simulink model "s_b4a4x1kf"  (R2018a)
settings: Solver=VariableStepDiscrete  StartTime=0.0  StopTime=1  RelTol=1e-3
undefined symbols (not defined in the file): fft_stages, n_bits_ants, n_bits_xengs
libraries: xbsIndex_r4 x22055, xbsReplacements_r4 x30, casper_library_misc x29, casper_library_scopes x15, xps_library x4
(part 89 of 227)

== system s_b4a4x1kf/sys3/vacc/vacc_time ==
  note: If we're going to relock,
      | lock two accs ahead.
      | (give VACCs chance to reset)
  note: If we were armed and somehow missed the
      | trigger, then re-arm.
      |
      | If we're waiting for a timestamp more than 2 accs ahead
      | (rew) of incoming timestamps, also re-arm.
      |
      | If an error occurs inside the VACC, also re-arm.
  note: If we detected an error,
      | wait 'till we've caught up to the incoming timestamp,
      | then rearm.
  note: fast-forward if we're
      | behind the incoming
      | timestamp.
  note: Rewind our record if we're more than
      | 2 accumulations ahead of incoming
      | timestampls.
  timestamp_in : Inport
  acc_len : Inport  Port=2
  valid_in : Inport  Port=3
  rb_done : Inport  Port=4
  arm : Inport  Port=5
  load_time : Inport  Port=6
  immediate : Inport  Port=7
  ext_err : Inport  Port=8
  AddSub : xbsIndex_r4/AddSub  mode=Subtraction  use_carryin=off  use_carryout=off  en=off  latency=1  precision=User Defined  arith_type=Unsigned  n_bits=timestamp_bits  bin_pt=0  quantization=Truncate  overflow=Wrap  use_behavioral_HDL=off  hw_selection=Fabric  pipelined=off  dbl_ovrd=off  block_type=addsub
  AddSub1 : xbsIndex_r4/AddSub  mode=Addition or Subtraction  use_carryin=off  use_carryout=off  en=on  latency=1  precision=User Defined  arith_type=Unsigned  n_bits=timestamp_bits  bin_pt=0  quantization=Truncate  overflow=Wrap  use_behavioral_HDL=on  hw_selection=Fabric  pipelined=off  dbl_ovrd=off  block_type=addsub
  AddSub2 : xbsIndex_r4/AddSub  mode=Addition  use_carryin=off  use_carryout=off  en=off  latency=1  precision=User Defined  arith_type=Unsigned  n_bits=timestamp_bits  bin_pt=0  quantization=Truncate  overflow=Wrap  use_behavioral_HDL=off  hw_selection=Fabric  pipelined=off  dbl_ovrd=off  block_type=addsub
  AddSub4 : xbsIndex_r4/AddSub  mode=Addition  use_carryin=off  use_carryout=off  en=off  latency=1  precision=User Defined  arith_type=Unsigned  n_bits=timestamp_bits  bin_pt=0  quantization=Truncate  overflow=Wrap  use_behavioral_HDL=off  hw_selection=Fabric  pipelined=off  dbl_ovrd=off  block_type=addsub
  Constant1 : xbsIndex_r4/Constant  const=0  gui_display_data_type=Fixed-point  arith_type=Unsigned  n_bits=1  bin_pt=0  preci_type=Single  exp_width=8  frac_width=24  explicit_period=on  period=1  equ=P=C  opselect=C  inp2=PCIN>>17  opr=+  inp1=P  carry=CIN  dbl_ovrd=off  block_type=constant
  Delay{7..10,13..14,23,26..29,32} (12 alike) : xbsIndex_r4/Delay  rst=off  infoeditControl=Selection of Reset will increase slice count due to use of real FFs and instead of SRLs  en=off  latency=1  reg_retiming=on  dbl_ovrd=off  block_type=delay
      Delay10 settings: infoedit=Hardware notes: A delay line is a chain, each link of which is an SRL16 or SRL32 followed by a flip-flop.
      Delay13 settings: infoedit=Hardware notes: A delay line is a chain, each link of which is an SRL16 or SRL32 followed by a flip-flop.
      Delay14 settings: infoedit=Hardware notes: A delay line is a chain, each link of which is an SRL16 or SRL32 followed by a flip-flop.
      Delay23 settings: infoedit=Hardware notes: A delay line is a chain, each link of which is an SRL16 or SRL32 followed by a flip-flop.
      Delay26 settings: infoedit=Hardware notes: A delay line is a chain, each link of which is an SRL16 or SRL32 followed by a flip-flop.
      Delay27 settings: infoedit=Hardware notes: A delay line is a chain, each link of which is an SRL16 or SRL32 followed by a flip-flop.
      Delay28 settings: infoedit=Hardware notes: A delay line is a chain, each link of which is an SRL16 or SRL32 followed by a flip-flop.
      Delay32 settings: infoedit=Hardware notes: A delay line is a chain, each link of which is an SRL16 or SRL32 followed by a flip-flop.
      Delay7 settings: infoedit=Hardware notes: A delay line is a chain, each link of which is an SRL16 or SRL32 followed by a flip-flop.
      Delay9 settings: infoedit=Hardware notes: A delay line is a chain, each link of which is an SRL16 or SRL32 followed by a flip-flop.
  Delay{15..16,19..22,30} (7 alike) : xbsIndex_r4/Delay  rst=off  infoeditControl=Selection of Reset will increase slice count due to use of real FFs and instead of SRLs  en=off  latency=2  reg_retiming=on  dbl_ovrd=off  block_type=delay
      settings: infoedit=Hardware notes: A delay line is a chain, each link of which is an SRL16 or SRL32 followed by a flip-flop.
  FIFO : xbsIndex_r4/FIFO  mem_type=Distributed RAM  performance_options=First_Word_Fall_Through  embedded_registers=off  depth=16  percent_nbits=1  rst=on  rst_latency=1  en=off  use_dcount=off  use_percent_full_port=off  use_almost_empty=off  almost_empty_thresh=2  use_almost_full=off  use_rd_rst_busy=off  use_wr_rst_busy=off  almost_full_thresh=14  explicit_period=off  dbl_ovrd=off  block_type=fifo
  Inverter{,1..3} (4 alike) : xbsIndex_r4/Inverter  en=off  latency=0  dbl_ovrd=off  block_type=inv
  Logical : xbsIndex_r4/Logical  logical_function=OR  inputs=3  en=off  latency=0  precision=Full  arith_type=Unsigned  n_bits=16  bin_pt=0  align_bp=on  dbl_ovrd=off  block_type=logical
  Logical{1,7,12..13} (4 alike) : xbsIndex_r4/Logical  logical_function=AND  inputs=2  en=off  latency=0  precision=Full  arith_type=Unsigned  n_bits=16  bin_pt=0  align_bp=on  dbl_ovrd=off  block_type=logical
  Logical10 : xbsIndex_r4/Logical  logical_function=OR  inputs=3  en=off  latency=0  precision=Full  arith_type=Unsigned  n_bits=16  bin_pt=0  align_bp=on  dbl_ovrd=off  block_type=logical
  Logical{4..5,9,11} (4 alike) : xbsIndex_r4/Logical  logical_function=OR  inputs=2  en=off  latency=0  precision=Full  arith_type=Unsigned  n_bits=16  bin_pt=0  align_bp=on  dbl_ovrd=off  block_type=logical
  Logical2 : xbsIndex_r4/Logical  logical_function=OR  inputs=4  en=off  latency=0  precision=Full  arith_type=Unsigned  n_bits=16  bin_pt=0  align_bp=on  dbl_ovrd=off  block_type=logical
  Logical3 : xbsIndex_r4/Logical  logical_function=AND  inputs=3  en=off  latency=0  precision=Full  arith_type=Unsigned  n_bits=16  bin_pt=0  align_bp=on  dbl_ovrd=off  block_type=logical
  Mux : xbsIndex_r4/Mux  inputs=2  en=off  latency=1  precision=Full  arith_type=Unsigned  n_bits=16  bin_pt=14  quantization=Truncate  overflow=Wrap  dbl_ovrd=off  block_type=mux
  Register{1..3,5} (4 alike) : xbsIndex_r4/Register  init=0  rst=off  en=on  dbl_ovrd=off  block_type=register
  Register4 : xbsIndex_r4/Register  init=0  rst=on  en=on  dbl_ovrd=off  block_type=register
  Relational : xbsIndex_r4/Relational  mode=a!=b  op_type=Bool  en=off  latency=1  dbl_ovrd=off  block_type=relational
  Relational1 : xbsIndex_r4/Relational  mode=a>b  op_type=Bool  en=off  latency=1  dbl_ovrd=off  block_type=relational
  Relational2 : xbsIndex_r4/Relational  mode=a=b  op_type=Bool  en=off  latency=1  dbl_ovrd=off  block_type=relational
      settings: block_version=10.1.3
  Relational3 : xbsIndex_r4/Relational  mode=a=b  op_type=Bool  en=off  latency=1  dbl_ovrd=off  block_type=relational
      settings: block_version=10.1.3
  Relational4 : xbsIndex_r4/Relational  mode=a!=b  op_type=Bool  en=off  latency=1  dbl_ovrd=off  block_type=relational
  Relational5 : xbsIndex_r4/Relational  mode=a<b  op_type=Bool  en=off  latency=1  dbl_ovrd=off  block_type=relational
  Relational6 : xbsIndex_r4/Relational  mode=a>b  op_type=Bool  en=off  latency=1  dbl_ovrd=off  block_type=relational
  Shift : xbsIndex_r4/Shift  shift_dir=Left  shift_bits=1  en=off  latency=0  precision=Full  arith_type="Signed  (2's comp)"  n_bits=16  bin_pt=14  quantization=Truncate  overflow=Wrap  dbl_ovrd=off  block_type=shift
  Shift2 : xbsIndex_r4/Shift  shift_dir=Left  shift_bits=1  en=off  latency=0  precision=Full  arith_type="Signed  (2's comp)"  n_bits=16  bin_pt=14  quantization=Truncate  overflow=Wrap  dbl_ovrd=off  block_type=shift
  armed_reg : xbsIndex_r4/Register  init=0  rst=on  en=on  dbl_ovrd=off  block_type=register
  edge_detect1 : Subsystem  mask(edge_detect){edge=Rising, polarity=Active High, x_in=[0 0.08 0.08 0.16 0.16 0.24 0.24 0.32 0.32 0.4], y_in=[-1 -1  1  1  1  1  1  1  1  1], x_out=[0.6 0.68 0.68 0.76 0.76 0.84 0.84 0.92 0.92 1], y_out=[-1 -1  1  1 -1 -1 -1 -1 -1 -1]}
      mask prompts: edge "Edge Type"; polarity "Output Polarity"; x_in "Input X Positions"; y_in "Input Y Positions"; x_out "Output X Positions"; y_out "Output Y Positions"
      mask help: Output is active for one-cycle after each edge of the specified type (i.e. rising, falling or both).
      mask init: same as s_b4a4x1kf/edge_detect
      settings: AttributesFormatString=|
      | rising edges
      | active high
      mask Help: Output is active for one-cycle after each edge of the specified type (i.e. rising, falling, or both).  Latency is zero.
      mask TypeOptions edge: Rising | Falling | Both
      mask TypeOptions polarity: Active High | Active Low
      mask Display:
      | plot(x_in_num,0.5+y_in_num*0.2);
      | plot(x_out_num,0.5+y_out_num*0.2);
  edge_detect2 : Subsystem  mask(edge_detect){edge=Rising, polarity=Active High, x_in=[0 0.08 0.08 0.16 0.16 0.24 0.24 0.32 0.32 0.4], y_in=[-1 -1  1  1  1  1  1  1  1  1], x_out=[0.6 0.68 0.68 0.76 0.76 0.84 0.84 0.92 0.92 1], y_out=[-1 -1  1  1 -1 -1 -1 -1 -1 -1]}
      mask prompts: edge "Edge Type"; polarity "Output Polarity"; x_in "Input X Positions"; y_in "Input Y Positions"; x_out "Output X Positions"; y_out "Output Y Positions"
      mask help: Output is active for one-cycle after each edge of the specified type (i.e. rising, falling or both).
      mask init: same as s_b4a4x1kf/edge_detect
      settings: AttributesFormatString=|
      | rising edges
      | active high
      mask Help: Output is active for one-cycle after each edge of the specified type (i.e. rising, falling, or both).  Latency is zero.
      mask TypeOptions edge: Rising | Falling | Both
      mask TypeOptions polarity: Active High | Active Low
      mask Display:
      | plot(x_in_num,0.5+y_in_num*0.2);
      | plot(x_out_num,0.5+y_out_num*0.2);
  edge_detect3 : Subsystem  mask(edge_detect){edge=Rising, polarity=Active High, x_in=[0 0.08 0.08 0.16 0.16 0.24 0.24 0.32 0.32 0.4], y_in=[-1 -1  1  1  1  1  1  1  1  1], x_out=[0.6 0.68 0.68 0.76 0.76 0.84 0.84 0.92 0.92 1], y_out=[-1 -1  1  1 -1 -1 -1 -1 -1 -1]}
      mask prompts: edge "Edge Type"; polarity "Output Polarity"; x_in "Input X Positions"; y_in "Input Y Positions"; x_out "Output X Positions"; y_out "Output Y Positions"
      mask help: Output is active for one-cycle after each edge of the specified type (i.e. rising, falling or both).
      mask init: same as s_b4a4x1kf/edge_detect
      settings: AttributesFormatString=|
      | rising edges
      | active high
      mask Help: Output is active for one-cycle after each edge of the specified type (i.e. rising, falling, or both).  Latency is zero.
      mask TypeOptions edge: Rising | Falling | Both
      mask TypeOptions polarity: Active High | Active Low
      mask Display:
      | plot(x_in_num,0.5+y_in_num*0.2);
      | plot(x_out_num,0.5+y_out_num*0.2);
  edge_detect4 : Subsystem  mask(edge_detect){edge=Rising, polarity=Active High, x_in=[0 0.08 0.08 0.16 0.16 0.24 0.24 0.32 0.32 0.4], y_in=[-1 -1  1  1  1  1  1  1  1  1], x_out=[0.6 0.68 0.68 0.76 0.76 0.84 0.84 0.92 0.92 1], y_out=[-1 -1  1  1 -1 -1 -1 -1 -1 -1]}
      mask prompts: edge "Edge Type"; polarity "Output Polarity"; x_in "Input X Positions"; y_in "Input Y Positions"; x_out "Output X Positions"; y_out "Output Y Positions"
      mask help: Output is active for one-cycle after each edge of the specified type (i.e. rising, falling or both).
      mask init: same as s_b4a4x1kf/edge_detect
      settings: AttributesFormatString=|
      | rising edges
      | active high
      mask Help: Output is active for one-cycle after each edge of the specified type (i.e. rising, falling, or both).  Latency is zero.
      mask TypeOptions edge: Rising | Falling | Both
      mask TypeOptions polarity: Active High | Active Low
      mask Display:
      | plot(x_in_num,0.5+y_in_num*0.2);
      | plot(x_out_num,0.5+y_out_num*0.2);
  edge_detect5 : Subsystem  mask(edge_detect){edge=Rising, polarity=Active High, x_in=[0 0.08 0.08 0.16 0.16 0.24 0.24 0.32 0.32 0.4], y_in=[-1 -1  1  1  1  1  1  1  1  1], x_out=[0.6 0.68 0.68 0.76 0.76 0.84 0.84 0.92 0.92 1], y_out=[-1 -1  1  1 -1 -1 -1 -1 -1 -1]}
      mask prompts: edge "Edge Type"; polarity "Output Polarity"; x_in "Input X Positions"; y_in "Input Y Positions"; x_out "Output X Positions"; y_out "Output Y Positions"
      mask help: Output is active for one-cycle after each edge of the specified type (i.e. rising, falling or both).
      mask init: same as s_b4a4x1kf/edge_detect
      settings: AttributesFormatString=|
      | rising edges
      | active high
      mask Help: Output is active for one-cycle after each edge of the specified type (i.e. rising, falling, or both).  Latency is zero.
      mask TypeOptions edge: Rising | Falling | Both
      mask TypeOptions polarity: Active High | Active Low
      mask Display:
      | plot(x_in_num,0.5+y_in_num*0.2);
      | plot(x_out_num,0.5+y_out_num*0.2);
  edge_detect6 : Subsystem  mask(edge_detect){edge=Rising, polarity=Active High, x_in=[0 0.08 0.08 0.16 0.16 0.24 0.24 0.32 0.32 0.4], y_in=[-1 -1  1  1  1  1  1  1  1  1], x_out=[0.6 0.68 0.68 0.76 0.76 0.84 0.84 0.92 0.92 1], y_out=[-1 -1  1  1 -1 -1 -1 -1 -1 -1]}
      mask prompts: edge "Edge Type"; polarity "Output Polarity"; x_in "Input X Positions"; y_in "Input Y Positions"; x_out "Output X Positions"; y_out "Output Y Positions"
      mask help: Output is active for one-cycle after each edge of the specified type (i.e. rising, falling or both).
      mask init: same as s_b4a4x1kf/edge_detect
      settings: AttributesFormatString=|
      | rising edges
      | active high
      mask Help: Output is active for one-cycle after each edge of the specified type (i.e. rising, falling, or both).  Latency is zero.
      mask TypeOptions edge: Rising | Falling | Both
      mask TypeOptions polarity: Active High | Active Low
      mask Display:
      | plot(x_in_num,0.5+y_in_num*0.2);
      | plot(x_out_num,0.5+y_out_num*0.2);
  edge_detect7 : Subsystem  mask(edge_detect){edge=Both, polarity=Active High, x_in=[0 0.08 0.08 0.16 0.16 0.24 0.24 0.32 0.32 0.4], y_in=[-1 -1  1  1  1  1  1  1  1  1], x_out=[0.6 0.68 0.68 0.76 0.76 0.84 0.84 0.92 0.92 1], y_out=[-1 -1  1  1 -1 -1 -1 -1 -1 -1]}
      mask prompts: edge "Edge Type"; polarity "Output Polarity"; x_in "Input X Positions"; y_in "Input Y Positions"; x_out "Output X Positions"; y_out "Output Y Positions"
      mask help: Output is active for one-cycle after each edge of the specified type (i.e. rising, falling or both).
      mask init: same as s_b4a4x1kf/edge_detect
      settings: AttributesFormatString=|
      | both edges
      | active high
      mask Help: Output is active for one-cycle after each edge of the specified type (i.e. rising, falling, or both).  Latency is zero.
      mask TypeOptions edge: Rising | Falling | Both
      mask TypeOptions polarity: Active High | Active Low
      mask Display:
      | plot(x_in_num,0.5+y_in_num*0.2);
      | plot(x_out_num,0.5+y_out_num*0.2);
  segment : Subsystem
  timestamp_out : Outport
  armed : Outport  Port=2
  acc_start : Outport  Port=3
  ts_err : Outport  Port=4
  wires:
  armed_reg/1 -> [armed]
  rb_done/1 -> edge_detect1/1(in)
  Register2/1 -> AddSub/2
  AddSub/1 -> Relational/1, Relational4/1
  [acc_len] -> Relational/2
  Delay7/1 -> AddSub1/2
  [armed] -> Delay20/1
  acc_len/1 -> [acc_len]
  [acc_len] -> segment/3(acc_len)
  [acc_len] -> Delay7/1
  Logical/1 -> armed_reg/2
  arm/1 -> edge_detect3/1(in)
  load_time/1 -> Register3/1
  Register3/1 -> [ext_load_time_latched], Relational2/2
  immediate/1 -> Delay32/1
  Relational2/1 -> edge_detect4/1(in)
  Delay8/1 -> edge_detect5/1(in)
  edge_detect4/1(out) -> Logical/1
  timestamp_in/1 -> Delay10/1, Relational3/1, Relational2/1
  [armed] -> segment/1(arm)
  [armed] -> armed/1
  [acc_start] -> Logical2/1
  Relational1/1 -> [ffwd]
  [ffwd] -> Logical2/2
  valid_in/1 -> Delay9/1
  [valid_in] -> segment/2(valid)
  Register4/1 -> [latched_err]
  [ffwd] -> Inverter/1
  [latched_err] -> Logical3/1
  Inverter/1 -> Logical3/2
  Relational3/1 -> edge_detect2/1(in)
  edge_detect2/1(out) -> Logical/2
  edge_detect5/1(out) -> Logical/3
  Logical4/1 -> [rearm], armed_reg/3, armed_reg/1
  [ext_arm] -> Logical4/2
  [relock_arm] -> edge_detect6/1(in)
  edge_detect6/1(out) -> Logical4/1
  [relock_ts] -> Mux/2
  Mux/1 -> AddSub1/1
  [ext_load_time_latched] -> Mux/3
  Inverter1/1 -> Logical3/3
  Logical11/1 -> Register1/2
  Delay9/1 -> Delay13/1
  Delay10/1 -> Delay14/1
  Delay13/1 -> [valid_in]
  Delay14/1 -> [ts_in]
  [ts_in] -> Delay15/1
  [valid_in] -> Delay16/1
  [armed] -> Delay22/1
  Delay19/1 -> Register1/1
  segment/1(acc_start) -> [acc_start]
  [ext_arm] -> Delay26/1
  [ext_arm] -> Mux/1
  Delay20/1 -> Logical11/2, Delay21/1
  Delay21/1 -> Logical5/2
  Logical5/1 -> Register2/2
  [acc_start] -> Logical5/1
  [acc_start] -> Logical11/1
  FIFO/1 -> [ts_out], timestamp_out/1
  edge_detect1/1(out) -> [rb_done]
  [ts_in] -> Delay19/1
  edge_detect3/1(out) -> Register3/2, Delay27/1
  [acc_start] -> acc_start/1
  [rb_done] -> FIFO/3
  [acc_start] -> Delay28/1
  [ts_in] -> Delay23/1
  [armed] -> FIFO/4
  Delay23/1 -> FIFO/1
  Delay28/1 -> FIFO/2
  Constant1/1 -> Relational4/2
  Relational/1 -> Logical1/1
  Relational4/1 -> Logical1/2
  Logical1/1 -> [ts_err]
  Register1/1 -> Register2/1, Delay29/1
  Delay29/1 -> AddSub/1
  Logical2/1 -> AddSub1/4
  Relational5/1 -> [rew]
  [rew] -> Logical2/4
  [rew] -> AddSub1/3
  [relock_ts] -> Relational5/2
  [ts_in] -> AddSub2/1
  AddSub2/1 -> Relational5/1
  [acc_len] -> Shift/1
  Shift/1 -> AddSub2/2
  Delay30/1 -> ts_err/1
  [rew] -> Inverter1/1
  [latched_relock_ts] -> Relational3/2
  Logical3/1 -> [relock_arm]
  Logical10/1 -> Register4/3, Register4/1
  [ts_err] -> Logical12/1
  [armed] -> Inverter2/1
  Inverter2/1 -> Logical12/2
  Logical12/1 -> Logical10/2
  [rearm] -> Register4/2
  [relock_ts] -> Relational1/2
  [ts_in] -> Relational1/1
  [latched_relock_ts] -> Relational6/2
  [ts_in] -> Relational6/1
  AddSub1/1 -> [relock_ts]
  [relock_arm] -> Register5/2
  Register5/1 -> [latched_relock_ts]
  Shift2/1 -> AddSub4/2
  [relock_ts] -> AddSub4/1
  [acc_len] -> Shift2/1
  AddSub4/1 -> Register5/1
  Logical7/1 -> Logical10/1
  [armed] -> Logical7/2
  Relational6/1 -> Logical9/1
  Logical9/1 -> Logical7/1
  [rew] -> Logical9/2
  Delay26/1 -> Logical2/3
  Delay27/1 -> [ext_arm]
  Delay32/1 -> Delay8/1
  Inverter3/1 -> Logical13/2
  [armed] -> Inverter3/1
  [ext_err] -> Logical13/1
  Logical13/1 -> Logical10/3
  ext_err/1 -> [ext_err]
  [latched_err] -> edge_detect7/1(in)
  edge_detect7/1(out) -> Delay30/1

== system s_b4a4x1kf/sys3/vacc_tvg0/bus_replicate1 ==
  in : Inport
  bussify : Subsystem  mask(bus_create){inputNum=8}
      mask prompts: inputNum "Number of inputs:"
      mask init:
      | bus_create_init(gcb,...
      |     'inputNum', inputNum);
  out : Outport
  wires:
  in/1 -> bussify/1(in1), bussify/2(in2), bussify/3(in3), bussify/4(in4), bussify/5(in5), bussify/6(in6), bussify/7(in7), bussify/8(in8)
  bussify/1(bus_out) -> out/1

== system s_b4a4x1kf/sys3/vacc_tvg0/bus_replicate2 ==
  in : Inport
  bussify : Subsystem  mask(bus_create){inputNum=8}
      mask prompts: inputNum "Number of inputs:"
      mask init:
      | bus_create_init(gcb,...
      |     'inputNum', inputNum);
  out : Outport
  wires:
  in/1 -> bussify/1(in1), bussify/2(in2), bussify/3(in3), bussify/4(in4), bussify/5(in5), bussify/6(in6), bussify/7(in7), bussify/8(in8)
  bussify/1(bus_out) -> out/1

== system s_b4a4x1kf/sys3/vacc_tvg0/edge_detect ==
  in : Inport
  Delay : xbsIndex_r4/Delay  rst=off  infoeditControl=Selection of Reset will increase slice count due to use of real FFs and instead of SRLs  en=off  latency=1  reg_retiming=off  dbl_ovrd=off  block_type=delay
      settings: xl_area=[0, 0, 0, 0, 0, 0, 0]
  Inverter : xbsIndex_r4/Inverter  en=off  latency=0  dbl_ovrd=off  block_type=inv
      settings: xl_area=[0, 0, 0, 0, 0, 0, 0]
  edge_op : xbsIndex_r4/Logical  logical_function=NOR  inputs=2  en=off  latency=0  precision=Full  arith_type=Unsigned  n_bits=8  bin_pt=2  align_bp=on  dbl_ovrd=off  block_type=logical
      settings: xl_area=[0, 0, 0, 0, 0, 0, 0]
  out : Outport
  wires:
  Delay/1 -> edge_op/2
  in/1 -> Delay/1, Inverter/1
  edge_op/1 -> out/1
  Inverter/1 -> edge_op/1

== system s_b4a4x1kf/sys3/vacc_tvg0/edge_detect4 ==
  in : Inport
  Delay : xbsIndex_r4/Delay  rst=off  infoeditControl=Selection of Reset will increase slice count due to use of real FFs and instead of SRLs  en=off  latency=1  reg_retiming=on  dbl_ovrd=off  block_type=delay
      settings: xl_area=[0, 0, 0, 0, 0, 0, 0]
  Inverter : xbsIndex_r4/Inverter  en=off  latency=0  dbl_ovrd=off  block_type=inv
      settings: xl_area=[0, 0, 0, 0, 0, 0, 0]
  edge_op : xbsIndex_r4/Logical  logical_function=NOR  inputs=2  en=off  latency=0  precision=Full  arith_type=Unsigned  n_bits=8  bin_pt=2  align_bp=on  dbl_ovrd=off  block_type=logical
      settings: xl_area=[0, 0, 0, 0, 0, 0, 0]
  out : Outport
  wires:
  Inverter/1 -> edge_op/1
  edge_op/1 -> out/1
  in/1 -> Inverter/1, Delay/1
  Delay/1 -> edge_op/2

== system s_b4a4x1kf/sys3/vacc_tvg0/generate_pulses ==
  run : Inport
  num_pulses : Inport  Port=2
  num_per_group : Inport  Port=3
  group period : Inport  Port=4
  Constant : xbsIndex_r4/Constant  const=777777  gui_display_data_type=Fixed-point  arith_type=Unsigned  n_bits=20  bin_pt=0  preci_type=Single  exp_width=8  frac_width=24  explicit_period=on  period=1  equ=P=C  opselect=C  inp2=PCIN>>17  opr=+  inp1=P  carry=CIN  dbl_ovrd=off  block_type=constant
  Gateway Out{1..8} (8 alike) : xbsIndex_r4/Gateway Out  inherit_from_input=off  hdl_port=off  rows=1  columns=1  UseAsDAC=off  DACChannel='1'  interface=None  automatic_assignment=on  address_offset=hex2dec('00')  intf_name=''  intf_description=''  timing_constraint=None  locs_specified=off  LOCs={}  io_standard={}  block_type=gatewayout
      settings: infoedit="Gateway out block.  Converts Xilinx fixed point inputs into ouputs of type Simulink integer, double, or fixed point.<P><P>Hardware notes:  In hardware these blocks become top level output ports or are discarded, depending on how they are configured."  xl_area=[0, 0, 0, 0, 0, 0, 0]  block_version=10.1.3
  Inverter : xbsIndex_r4/Inverter  en=off  latency=0  dbl_ovrd=off  block_type=inv
  Logical1 : xbsIndex_r4/Logical  logical_function=AND  inputs=2  en=off  latency=0  precision=Full  arith_type=Unsigned  n_bits=8  bin_pt=2  align_bp=on  dbl_ovrd=off  block_type=logical
      settings: xl_area=[0, 0, 0, 0, 0, 0, 0]
  Logical2 : xbsIndex_r4/Logical  logical_function=AND  inputs=3  en=off  latency=0  precision=Full  arith_type=Unsigned  n_bits=8  bin_pt=2  align_bp=on  dbl_ovrd=off  block_type=logical
      settings: xl_area=[0, 0, 0, 0, 0, 0, 0]
  Logical3 : xbsIndex_r4/Logical  logical_function=AND  inputs=3  en=off  latency=0  precision=Full  arith_type=Unsigned  n_bits=8  bin_pt=2  align_bp=on  dbl_ovrd=off  block_type=logical
      settings: xl_area=[0, 0, 0, 0, 0, 0, 0]
  Logical4 : xbsIndex_r4/Logical  logical_function=OR  inputs=2  en=off  latency=0  precision=Full  arith_type=Unsigned  n_bits=8  bin_pt=2  align_bp=off  dbl_ovrd=off  block_type=logical
      settings: xl_area=[0, 0, 0, 0, 0, 0, 0]
  Logical5 : xbsIndex_r4/Logical  logical_function=OR  inputs=2  en=off  latency=0  precision=Full  arith_type=Unsigned  n_bits=8  bin_pt=2  align_bp=on  dbl_ovrd=off  block_type=logical
      settings: xl_area=[0, 0, 0, 0, 0, 0, 0]
  Logical6 : xbsIndex_r4/Logical  logical_function=AND  inputs=2  en=off  latency=0  precision=Full  arith_type=Unsigned  n_bits=8  bin_pt=2  align_bp=on  dbl_ovrd=off  block_type=logical
      settings: xl_area=[0, 0, 0, 0, 0, 0, 0]
  Relational : xbsIndex_r4/Relational  mode=a>=b  op_type=Bool  en=off  latency=0  dbl_ovrd=off  block_type=relational
      settings: xl_area=[0, 0, 0, 0, 0, 0, 0]  block_version=10.1.3
  Relational1 : xbsIndex_r4/Relational  mode=a=b  op_type=Bool  en=off  latency=0  dbl_ovrd=off  block_type=relational
      settings: xl_area=[0, 0, 0, 0, 0, 0, 0]  block_version=10.1.3
  Relational2 : xbsIndex_r4/Relational  mode=a>b  op_type=Bool  en=off  latency=0  dbl_ovrd=off  block_type=relational
      settings: xl_area=[0, 0, 0, 0, 0, 0, 0]  block_version=10.1.3
  Relational3 : xbsIndex_r4/Relational  mode=a=b  op_type=Bool  en=off  latency=0  dbl_ovrd=off  block_type=relational
      settings: xl_area=[0, 0, 0, 0, 0, 0, 0]  block_version=10.1.3
  Scope1 : Scope  NumInputPorts=4
  Scope2 : Scope  NumInputPorts=4
  edge_detect : Subsystem  mask(edge_detect){edge=Rising, polarity=Active High, x_in=[0 0.08 0.08 0.16 0.16 0.24 0.24 0.32 0.32 0.4], y_in=[-1 -1  1  1  1  1  1  1  1  1], x_out=[0.6 0.68 0.68 0.76 0.76 0.84 0.84 0.92 0.92 1], y_out=[-1 -1  1  1 -1 -1 -1 -1 -1 -1]}
      mask prompts: edge "Edge Type"; polarity "Output Polarity"; x_in "Input X Positions"; y_in "Input Y Positions"; x_out "Output X Positions"; y_out "Output Y Positions"
      mask help: Output is active for one-cycle after each edge of the specified type (i.e. rising, falling or both).
      mask init: same as s_b4a4x1kf/edge_detect
      settings: AttributesFormatString=|
      | rising edges
      | active high
      mask Help: Output is active for one-cycle after each edge of the specified type (i.e. rising, falling, or both).  Latency is zero.
      mask TypeOptions edge: Rising | Falling | Both
      mask TypeOptions polarity: Active High | Active Low
      mask Display:
      | plot(x_in_num,0.5+y_in_num*0.2);
      | plot(x_out_num,0.5+y_out_num*0.2);
  group_cntr : xbsIndex_r4/Counter  cnt_type=Free Running  cnt_to=1  operation=Up  start_count=1  cnt_by_val=1  arith_type=Unsigned  n_bits=32  bin_pt=0  load_pin=off  rst=on  en=off  explicit_period=on  period=1  use_behavioral_HDL=off  implementation=Fabric  use_rpm=on  dbl_ovrd=off  block_type=counter
      settings: xl_area=[0, 0, 0, 0, 0, 0, 0]
  pulse_cntr : xbsIndex_r4/Counter  cnt_type=Free Running  cnt_to=1  operation=Up  start_count=0  cnt_by_val=1  arith_type=Unsigned  n_bits=32  bin_pt=0  load_pin=off  rst=on  en=on  explicit_period=on  period=1  use_behavioral_HDL=off  implementation=Fabric  use_rpm=on  dbl_ovrd=off  block_type=counter
      settings: xl_area=[0, 0, 0, 0, 0, 0, 0]
  tot_cntr : xbsIndex_r4/Counter  cnt_type=Free Running  cnt_to=1  operation=Up  start_count=1  cnt_by_val=1  arith_type=Unsigned  n_bits=32  bin_pt=0  load_pin=off  rst=on  en=on  explicit_period=on  period=1  use_behavioral_HDL=off  implementation=Fabric  use_rpm=on  dbl_ovrd=off  block_type=counter
      settings: xl_area=[0, 0, 0, 0, 0, 0, 0]
  valid : Outport
  running : Outport  Port=2
  wires:
  tot_cntr/1 -> Relational/2, Gateway Out1/1
  run/1 -> Logical3/3, Logical2/1, Gateway Out8/1, edge_detect/1(in)
  Logical5/1 -> running/1, Logical2/3, Logical3/1, Gateway Out2/1, Logical1/2
  num_pulses/1 -> Relational/1, Relational3/1
  edge_detect/1(out) -> tot_cntr/1, Gateway Out3/1, Logical4/1
  group_cntr/1 -> Relational1/2, Gateway Out5/1
  Relational1/1 -> Logical4/2
  pulse_cntr/1 -> Relational2/2, Gateway Out4/1
  Relational2/1 -> Logical2/2
  num_per_group/1 -> Relational2/1
  Logical2/1 -> Gateway Out7/1, Logical6/1, pulse_cntr/2
  Logical4/1 -> Inverter/1, pulse_cntr/1, group_cntr/1
  group period/1 -> Relational1/1
  Gateway Out5/1 -> Scope2/3
  Gateway Out4/1 -> Scope2/2
  Gateway Out6/1 -> Scope2/1
  Gateway Out1/1 -> Scope2/4
  Gateway Out7/1 -> Scope1/3
  Gateway Out3/1 -> Scope1/2
  Gateway Out8/1 -> Scope1/1
  Gateway Out2/1 -> Scope1/4
  Logical6/1 -> Logical3/2, Logical1/1
  Logical1/1 -> Gateway Out6/1, valid/1
  Logical3/1 -> tot_cntr/2
  Constant/1 -> Relational3/2
  Relational/1 -> Logical5/1
  Relational3/1 -> Logical5/2
  Inverter/1 -> Logical6/2

== system s_b4a4x1kf/sys3/vacc_tvg0/generate_time ==
  sync_in : Inport
  din : Inport  Port=2
  valid_in : Inport  Port=3
  time_tvg_en : Inport  Port=4
  time_in : Inport  Port=5
  offset : Inport  Port=6
  AddSub : xbsIndex_r4/AddSub  mode=Addition  use_carryin=off  use_carryout=off  en=off  latency=1  precision=User Defined  arith_type=Unsigned  n_bits=time_bits  bin_pt=0  quantization=Truncate  overflow=Wrap  use_behavioral_HDL=off  hw_selection=Fabric  pipelined=off  dbl_ovrd=off  block_type=addsub
  Delay1 : xbsIndex_r4/Delay  rst=off  infoeditControl=Selection of Reset will increase slice count due to use of real FFs and instead of SRLs  en=off  latency=1  reg_retiming=on  dbl_ovrd=off  block_type=delay
      settings: xl_area=[0, 0, 0, 0, 0, 0, 0]
  Delay{2..3,9,13} (4 alike) : xbsIndex_r4/Delay  rst=off  infoeditControl=Selection of Reset will increase slice count due to use of real FFs and instead of SRLs  en=off  latency=2  reg_retiming=on  dbl_ovrd=off  block_type=delay
  Delay6 : xbsIndex_r4/Delay  rst=off  infoeditControl=Selection of Reset will increase slice count due to use of real FFs and instead of SRLs  en=off  latency=1  reg_retiming=on  dbl_ovrd=off  block_type=delay
      settings: xl_area=[0, 0, 0, 0, 0, 0, 0]
  Delay8 : xbsIndex_r4/Delay  rst=off  infoeditControl=Selection of Reset will increase slice count due to use of real FFs and instead of SRLs  en=off  latency=1  reg_retiming=on  dbl_ovrd=off  block_type=delay
      settings: xl_area=[0, 0, 0, 0, 0, 0, 0]
  Mux4 : xbsIndex_r4/Mux  inputs=2  en=off  latency=0  precision=Full  arith_type="Signed  (2's comp)"  n_bits=8  bin_pt=2  quantization=Truncate  overflow=Wrap  dbl_ovrd=off  block_type=mux
      settings: xl_area=[0, 0, 0, 0, 0, 0, 0]
  edge_detect1 : Subsystem  mask(edge_detect){edge=Rising, polarity=Active High, x_in=[0 0.08 0.08 0.16 0.16 0.24 0.24 0.32 0.32 0.4], y_in=[-1 -1  1  1  1  1  1  1  1  1], x_out=[0.6 0.68 0.68 0.76 0.76 0.84 0.84 0.92 0.92 1], y_out=[-1 -1  1  1 -1 -1 -1 -1 -1 -1]}
      mask prompts: edge "Edge Type"; polarity "Output Polarity"; x_in "Input X Positions"; y_in "Input Y Positions"; x_out "Output X Positions"; y_out "Output Y Positions"
      mask help: Output is active for one-cycle after each edge of the specified type (i.e. rising, falling or both).
      mask init: same as s_b4a4x1kf/edge_detect
      settings: AttributesFormatString=|
      | rising edges
      | active high
      mask Help: Output is active for one-cycle after each edge of the specified type (i.e. rising, falling, or both).  Latency is zero.
      mask TypeOptions edge: Rising | Falling | Both
      mask TypeOptions polarity: Active High | Active Low
      mask Display:
      | plot(x_in_num,0.5+y_in_num*0.2);
      | plot(x_out_num,0.5+y_out_num*0.2);
  group_cntr1 : xbsIndex_r4/Counter  cnt_type=Free Running  cnt_to=1  operation=Up  start_count=0  cnt_by_val=1  arith_type=Unsigned  n_bits=time_bits  bin_pt=0  load_pin=off  rst=on  en=on  explicit_period=on  period=1  use_behavioral_HDL=off  implementation=Fabric  use_rpm=on  dbl_ovrd=off  block_type=counter
      settings: xl_area=[0, 0, 0, 0, 0, 0, 0]
  segment : Subsystem
  sync_out : Outport
  dout : Outport  Port=2
  valid_out : Outport  Port=3
  time_out : Outport  Port=4
  wires:
  Delay1/1 -> dout/1
  Delay8/1 -> valid_out/1
  Delay6/1 -> sync_out/1
  AddSub/1 -> time_out/1
  group_cntr1/1 -> Mux4/3
  segment/1(vector_start) -> group_cntr1/2
  Delay13/1 -> Delay8/1
  Delay9/1 -> Mux4/2
  Mux4/1 -> AddSub/1
  time_tvg_en/1 -> Mux4/1, edge_detect1/1(in)
  offset/1 -> AddSub/2
  sync_in/1 -> Delay3/1, segment/1(sync_in)
  valid_in/1 -> segment/2(valid), Delay13/1
  edge_detect1/1(out) -> group_cntr1/1
  din/1 -> Delay2/1
  Delay2/1 -> Delay1/1
  time_in/1 -> Delay9/1
  Delay3/1 -> Delay6/1

== system s_b4a4x1kf/sys3/vacc_tvg0/group_period ==
  sim_1 : Inport
  convert1_1 : DataTypeConversion  OutDataTypeStr=fixdt('ufix32_En0')  LockScale=on
  convert2_1 : DataTypeConversion  OutDataTypeStr=fixdt('ufix32_En0')  ConvertRealWorld=Stored Integer (SI)  LockScale=on
  gain_1 : Gain
  io_delay : xbsIndex_r4/Delay  rst=off  infoeditControl=Selection of Reset will increase slice count due to use of real FFs and instead of SRLs  en=off  latency=0  reg_retiming=on  dbl_ovrd=off  block_type=delay
  reint1 : xbsIndex_r4/Reinterpret  force_arith_type=on  arith_type=Unsigned  force_bin_pt=on  bin_pt=0  block_type=reinterpret
  s_b4a4x1kf_sys3_vacc_tvg0_group_period_user_data_out : xbsIndex_r4/Gateway In  gui_display_data_type=Fixed-point  arith_type=Unsigned  n_bits=32  bin_pt=0  preci_type=Single  exp_width=8  frac_width=24  rows=1  columns=1  quantization="Round  (unbiased: +/- Inf)"  overflow=Saturate  period=1  UseAsADC=off  ADCChannel='1'  interface=None  automatic_assignment=on  address_offset=hex2dec('00')  intf_name=''  intf_description=''  default_value=0  timing_constraint=None  locs_specified=off  LOCs={}  io_standard={}  inherit_from_input=off  hdl_port=on  dbl_ovrd=off  block_type=gatewayin
  slice_reg : xbsIndex_r4/Slice  nbits=32  boolean_output=off  mode=Lower Bit Location + Width  bit1=0  base1=MSB of Input  bit0=0  base0=LSB of Input  dbl_ovrd=off  block_type=slice
  in_reg : Outport
  wires:
  s_b4a4x1kf_sys3_vacc_tvg0_group_period_user_data_out/1 -> io_delay/1
  sim_1/1 -> convert1_1/1
  convert1_1/1 -> convert2_1/1
  convert2_1/1 -> gain_1/1
  gain_1/1 -> s_b4a4x1kf_sys3_vacc_tvg0_group_period_user_data_out/1
  io_delay/1 -> slice_reg/1
  slice_reg/1 -> reint1/1
  reint1/1 -> in_reg/1

== system s_b4a4x1kf/sys3/vacc_tvg0/ins_counter ==
  new_acc_in : Inport
  din : Inport  Port=2
  valid_in : Inport  Port=3
  enable : Inport  Port=4
  misci : Inport  Port=5
  Counter : xbsIndex_r4/Counter  cnt_type=Count Limited  cnt_to=vec_len-1  operation=Up  start_count=0  cnt_by_val=1  arith_type=Unsigned  n_bits=n_bits  bin_pt=0  load_pin=off  rst=on  en=on  explicit_period=off  period=1  use_behavioral_HDL=off  implementation=Fabric  use_rpm=on  dbl_ovrd=off  block_type=counter
      settings: xl_area=[0, 0, 0, 0, 0, 0, 0]
  Delay{,1..6} (7 alike) : xbsIndex_r4/Delay  rst=off  infoeditControl=Selection of Reset will increase slice count due to use of real FFs and instead of SRLs  en=off  latency=1  reg_retiming=on  dbl_ovrd=off  block_type=delay
      settings: xl_area=[0, 0, 0, 0, 0, 0, 0]
  Gateway Out4 : xbsIndex_r4/Gateway Out  inherit_from_input=off  hdl_port=off  rows=1  columns=1  UseAsDAC=off  DACChannel='1'  interface=None  automatic_assignment=on  address_offset=hex2dec('00')  intf_name=''  intf_description=''  timing_constraint=None  locs_specified=off  LOCs={}  io_standard={}  block_type=gatewayout
      settings: infoedit="Gateway out block.  Converts Xilinx fixed point inputs into ouputs of type Simulink integer, double, or fixed point.<P><P>Hardware notes:  In hardware these blocks become top level output ports or are discarded, depending on how they are configured."  xl_area=[0, 0, 0, 0, 0, 0, 0]  block_version=10.1.3
  Gateway Out5 : xbsIndex_r4/Gateway Out  inherit_from_input=off  hdl_port=off  rows=1  columns=1  UseAsDAC=off  DACChannel='1'  interface=None  automatic_assignment=on  address_offset=hex2dec('00')  intf_name=''  intf_description=''  timing_constraint=None  locs_specified=off  LOCs={}  io_standard={}  block_type=gatewayout
      settings: infoedit="Gateway out block.  Converts Xilinx fixed point inputs into ouputs of type Simulink integer, double, or fixed point.<P><P>Hardware notes:  In hardware these blocks become top level output ports or are discarded, depending on how they are configured."  xl_area=[0, 0, 0, 0, 0, 0, 0]  block_version=10.1.3
  Gateway Out6 : xbsIndex_r4/Gateway Out  inherit_from_input=off  hdl_port=off  rows=1  columns=1  UseAsDAC=off  DACChannel='1'  interface=None  automatic_assignment=on  address_offset=hex2dec('00')  intf_name=''  intf_description=''  timing_constraint=None  locs_specified=off  LOCs={}  io_standard={}  block_type=gatewayout
      settings: infoedit="Gateway out block.  Converts Xilinx fixed point inputs into ouputs of type Simulink integer, double, or fixed point.<P><P>Hardware notes:  In hardware these blocks become top level output ports or are discarded, depending on how they are configured."  xl_area=[0, 0, 0, 0, 0, 0, 0]  block_version=10.1.3
  Mux : xbsIndex_r4/Mux  inputs=2  en=off  latency=0  precision=Full  arith_type="Signed  (2's comp)"  n_bits=8  bin_pt=2  quantization=Truncate  overflow=Wrap  dbl_ovrd=off  block_type=mux
      settings: xl_area=[0, 0, 0, 0, 0, 0, 0]
  Scope2 : Scope  NumInputPorts=3
  bus_replicate1 : Subsystem  Tag=cmac_delinked  mask(bus_replicate){replication=n_inputs, csp_latency=0, misc=off, implementation=core}
      mask prompts: replication "replication factor"; csp_latency "latency"; misc "misc support"; implementation "delay implementation"
      mask help: Output bus formed by replicating input bus a number of times
      mask init:
      | bus_replicate_init(gcb, ...
      |     'replication', replication, ...
      |     'csp_latency', csp_latency, ...
      |     'implementation', implementation, ...
      |     'misc', misc);
      mask TypeOptions implementation: core | behavioral
  new_acc_out : Outport
  dout : Outport  Port=2
  valid_out : Outport  Port=3
  misco : Outport  Port=4
  wires:
  Delay5/1 -> Mux/1
  Delay4/1 -> Counter/1, Gateway Out6/1
  new_acc_in/1 -> Delay/1, Delay4/1
  valid_in/1 -> Delay1/1, Delay3/1
  enable/1 -> Delay5/1
  din/1 -> Delay2/1
  Counter/1 -> bus_replicate1/1(in)
  Mux/1 -> dout/1
  Delay/1 -> new_acc_out/1
  Delay1/1 -> valid_out/1
  Delay2/1 -> Mux/2
  Gateway Out5/1 -> Scope2/3
  Gateway Out4/1 -> Scope2/2
  Gateway Out6/1 -> Scope2/1
  Delay3/1 -> Counter/2, Gateway Out5/1
  bus_replicate1/1(out) -> Mux/3, Gateway Out4/1
  misci/1 -> Delay6/1
  Delay6/1 -> misco/1

== system s_b4a4x1kf/sys3/vacc_tvg0/ins_counter2 ==
  sync_in : Inport
  din : Inport  Port=2
  valid_in : Inport  Port=3
  cnt_tvg_en : Inport  Port=4
  time_in : Inport  Port=5
  cnt_rst : Inport  Port=6
  Counter : xbsIndex_r4/Counter  cnt_type=Free Running  cnt_to=1  operation=Up  start_count=0  cnt_by_val=1  arith_type=Unsigned  n_bits=n_bits  bin_pt=0  load_pin=off  rst=on  en=on  explicit_period=off  period=1  use_behavioral_HDL=off  implementation=Fabric  use_rpm=on  dbl_ovrd=off  block_type=counter
      settings: xl_area=[0, 0, 0, 0, 0, 0, 0]
  Delay{1,3,6,8} (4 alike) : xbsIndex_r4/Delay  rst=off  infoeditControl=Selection of Reset will increase slice count due to use of real FFs and instead of SRLs  en=off  latency=1  reg_retiming=on  dbl_ovrd=off  block_type=delay
      settings: xl_area=[0, 0, 0, 0, 0, 0, 0]
  Delay{2,4..5,13} (4 alike) : xbsIndex_r4/Delay  rst=off  infoeditControl=Selection of Reset will increase slice count due to use of real FFs and instead of SRLs  en=off  latency=2  reg_retiming=on  dbl_ovrd=off  block_type=delay
  Mux : xbsIndex_r4/Mux  inputs=2  en=off  latency=0  precision=Full  arith_type="Signed  (2's comp)"  n_bits=8  bin_pt=2  quantization=Truncate  overflow=Wrap  dbl_ovrd=off  block_type=mux
      settings: xl_area=[0, 0, 0, 0, 0, 0, 0]
  bus_replicate1 : Subsystem  Tag=cmac_delinked  mask(bus_replicate){replication=n_inputs, csp_latency=0, misc=off, implementation=core}
      mask prompts: replication "replication factor"; csp_latency "latency"; misc "misc support"; implementation "delay implementation"
      mask help: Output bus formed by replicating input bus a number of times
      mask init:
      | bus_replicate_init(gcb, ...
      |     'replication', replication, ...
      |     'csp_latency', csp_latency, ...
      |     'implementation', implementation, ...
      |     'misc', misc);
      mask TypeOptions implementation: core | behavioral
  edge_detect : Subsystem  mask(edge_detect){edge=Rising, polarity=Active High, x_in=[0 0.08 0.08 0.16 0.16 0.24 0.24 0.32 0.32 0.4], y_in=[-1 -1  1  1  1  1  1  1  1  1], x_out=[0.6 0.68 0.68 0.76 0.76 0.84 0.84 0.92 0.92 1], y_out=[-1 -1  1  1 -1 -1 -1 -1 -1 -1]}
      mask prompts: edge "Edge Type"; polarity "Output Polarity"; x_in "Input X Positions"; y_in "Input Y Positions"; x_out "Output X Positions"; y_out "Output Y Positions"
      mask help: Output is active for one-cycle after each edge of the specified type (i.e. rising, falling or both).
      mask init: same as s_b4a4x1kf/edge_detect
      settings: AttributesFormatString=|
      | rising edges
      | active high
      mask Help: Output is active for one-cycle after each edge of the specified type (i.e. rising, falling, or both).  Latency is zero.
      mask TypeOptions edge: Rising | Falling | Both
      mask TypeOptions polarity: Active High | Active Low
      mask Display:
      | plot(x_in_num,0.5+y_in_num*0.2);
      | plot(x_out_num,0.5+y_out_num*0.2);
  segment : Subsystem
  sync_out : Outport
  dout : Outport  Port=2
  valid_out : Outport  Port=3
  time_out : Outport  Port=4
  wires:
  bus_replicate1/1(out) -> Mux/3
  Delay2/1 -> Mux/2
  Mux/1 -> Delay1/1
  Counter/1 -> bus_replicate1/1(in)
  din/1 -> Delay2/1
  cnt_tvg_en/1 -> Mux/1
  valid_in/1 -> Delay13/1, segment/2(valid)
  sync_in/1 -> segment/1(sync_in), Delay5/1
  Delay13/1 -> Delay8/1
  Delay6/1 -> sync_out/1
  Delay8/1 -> valid_out/1
  Delay1/1 -> dout/1
  edge_detect/1(out) -> Counter/1
  segment/1(vector_start) -> Counter/2
  time_in/1 -> Delay4/1
  Delay3/1 -> time_out/1
  Delay4/1 -> Delay3/1
  cnt_rst/1 -> edge_detect/1(in)
  Delay5/1 -> Delay6/1

== system s_b4a4x1kf/sys3/vacc_tvg0/ins_counter3 ==
  sync_in : Inport
  din : Inport  Port=2
  valid_in : Inport  Port=3
  cnt_tvg_en : Inport  Port=4
  time_in : Inport  Port=5
  cnt_rst : Inport  Port=6
  acc_len : Inport  Port=7
  Delay{1,3,6,8} (4 alike) : xbsIndex_r4/Delay  rst=off  infoeditControl=Selection of Reset will increase slice count due to use of real FFs and instead of SRLs  en=off  latency=1  reg_retiming=on  dbl_ovrd=off  block_type=delay
      settings: xl_area=[0, 0, 0, 0, 0, 0, 0]
  Delay{2,4..5,13} (4 alike) : xbsIndex_r4/Delay  rst=off  infoeditControl=Selection of Reset will increase slice count due to use of real FFs and instead of SRLs  en=off  latency=2  reg_retiming=on  dbl_ovrd=off  block_type=delay
  Logical7 : xbsIndex_r4/Logical  logical_function=OR  inputs=2  en=off  latency=0  precision=Full  arith_type=Unsigned  n_bits=16  bin_pt=0  align_bp=on  dbl_ovrd=off  block_type=logical
  Mux : xbsIndex_r4/Mux  inputs=2  en=off  latency=0  precision=Full  arith_type="Signed  (2's comp)"  n_bits=8  bin_pt=2  quantization=Truncate  overflow=Wrap  dbl_ovrd=off  block_type=mux
      settings: xl_area=[0, 0, 0, 0, 0, 0, 0]
  Relational1 : xbsIndex_r4/Relational  mode=a>=b  op_type=Bool  en=off  latency=0  dbl_ovrd=off  block_type=relational
      settings: block_version=10.1.3
  acc_cnt : xbsIndex_r4/Counter  cnt_type=Free Running  cnt_to=Inf  operation=Up  start_count=0  cnt_by_val=1  arith_type=Unsigned  n_bits=n_bits  bin_pt=0  load_pin=off  rst=on  en=on  explicit_period=on  period=1  use_behavioral_HDL=off  implementation=Fabric  use_rpm=off  dbl_ovrd=off  block_type=counter
  bus_replicate1 : Subsystem  Tag=cmac_delinked  mask(bus_replicate){replication=n_inputs, csp_latency=0, misc=off, implementation=core}
      mask prompts: replication "replication factor"; csp_latency "latency"; misc "misc support"; implementation "delay implementation"
      mask help: Output bus formed by replicating input bus a number of times
      mask init:
      | bus_replicate_init(gcb, ...
      |     'replication', replication, ...
      |     'csp_latency', csp_latency, ...
      |     'implementation', implementation, ...
      |     'misc', misc);
      mask TypeOptions implementation: core | behavioral
  edge_detect : Subsystem  mask(edge_detect){edge=Rising, polarity=Active High, x_in=[0 0.08 0.08 0.16 0.16 0.24 0.24 0.32 0.32 0.4], y_in=[-1 -1  1  1  1  1  1  1  1  1], x_out=[0.6 0.68 0.68 0.76 0.76 0.84 0.84 0.92 0.92 1], y_out=[-1 -1  1  1 -1 -1 -1 -1 -1 -1]}
      mask prompts: edge "Edge Type"; polarity "Output Polarity"; x_in "Input X Positions"; y_in "Input Y Positions"; x_out "Output X Positions"; y_out "Output Y Positions"
      mask help: Output is active for one-cycle after each edge of the specified type (i.e. rising, falling or both).
      mask init: same as s_b4a4x1kf/edge_detect
      settings: AttributesFormatString=|
      | rising edges
      | active high
      mask Help: Output is active for one-cycle after each edge of the specified type (i.e. rising, falling, or both).  Latency is zero.
      mask TypeOptions edge: Rising | Falling | Both
      mask TypeOptions polarity: Active High | Active Low
      mask Display:
      | plot(x_in_num,0.5+y_in_num*0.2);
      | plot(x_out_num,0.5+y_out_num*0.2);
  segment : Subsystem
  vect_cnt : xbsIndex_r4/Counter  cnt_type=Free Running  cnt_to=1  operation=Up  start_count=0  cnt_by_val=1  arith_type=Unsigned  n_bits=32  bin_pt=0  load_pin=off  rst=on  en=on  explicit_period=off  period=1  use_behavioral_HDL=off  implementation=Fabric  use_rpm=on  dbl_ovrd=off  block_type=counter
      settings: xl_area=[0, 0, 0, 0, 0, 0, 0]
  sync_out : Outport
  dout : Outport  Port=2
  valid_out : Outport  Port=3
  time_out : Outport  Port=4
  wires:
  cnt_rst/1 -> edge_detect/1(in)
  Delay4/1 -> Delay3/1
  Delay3/1 -> time_out/1
  time_in/1 -> Delay4/1
  segment/1(vector_start) -> vect_cnt/2
  Delay1/1 -> dout/1
  Delay8/1 -> valid_out/1
  Delay6/1 -> sync_out/1
  Delay13/1 -> Delay8/1
  sync_in/1 -> Delay5/1, segment/1(sync_in)
  valid_in/1 -> Delay13/1, segment/2(valid)
  cnt_tvg_en/1 -> Mux/1
  din/1 -> Delay2/1
  Mux/1 -> Delay1/1
  Delay2/1 -> Mux/2
  bus_replicate1/1(out) -> Mux/3
  vect_cnt/1 -> Relational1/1
  acc_cnt/1 -> bus_replicate1/1(in)
  edge_detect/1(out) -> Logical7/2, acc_cnt/1
  Relational1/1 -> Logical7/1, acc_cnt/2
  Logical7/1 -> vect_cnt/1
  acc_len/1 -> Relational1/2
  Delay5/1 -> Delay6/1

== system s_b4a4x1kf/sys3/vacc_tvg0/ins_vect_loc ==
  sim_1 : Inport
  convert1_1 : DataTypeConversion  OutDataTypeStr=fixdt('ufix32_En0')  LockScale=on
  convert2_1 : DataTypeConversion  OutDataTypeStr=fixdt('ufix32_En0')  ConvertRealWorld=Stored Integer (SI)  LockScale=on
  gain_1 : Gain
  io_delay : xbsIndex_r4/Delay  rst=off  infoeditControl=Selection of Reset will increase slice count due to use of real FFs and instead of SRLs  en=off  latency=0  reg_retiming=on  dbl_ovrd=off  block_type=delay
  reint1 : xbsIndex_r4/Reinterpret  force_arith_type=on  arith_type=Unsigned  force_bin_pt=on  bin_pt=0  block_type=reinterpret
  s_b4a4x1kf_sys3_vacc_tvg0_ins_vect_loc_user_data_out : xbsIndex_r4/Gateway In  gui_display_data_type=Fixed-point  arith_type=Unsigned  n_bits=32  bin_pt=0  preci_type=Single  exp_width=8  frac_width=24  rows=1  columns=1  quantization="Round  (unbiased: +/- Inf)"  overflow=Saturate  period=1  UseAsADC=off  ADCChannel='1'  interface=None  automatic_assignment=on  address_offset=hex2dec('00')  intf_name=''  intf_description=''  default_value=0  timing_constraint=None  locs_specified=off  LOCs={}  io_standard={}  inherit_from_input=off  hdl_port=on  dbl_ovrd=off  block_type=gatewayin
  slice_reg : xbsIndex_r4/Slice  nbits=32  boolean_output=off  mode=Lower Bit Location + Width  bit1=0  base1=MSB of Input  bit0=0  base0=LSB of Input  dbl_ovrd=off  block_type=slice
  in_reg : Outport
  wires:
  s_b4a4x1kf_sys3_vacc_tvg0_ins_vect_loc_user_data_out/1 -> io_delay/1
  sim_1/1 -> convert1_1/1
  convert1_1/1 -> convert2_1/1
  convert2_1/1 -> gain_1/1
  gain_1/1 -> s_b4a4x1kf_sys3_vacc_tvg0_ins_vect_loc_user_data_out/1
  io_delay/1 -> slice_reg/1
  slice_reg/1 -> reint1/1
  reint1/1 -> in_reg/1

== system s_b4a4x1kf/sys3/vacc_tvg0/ins_vect_val ==
  sim_1 : Inport
  convert1_1 : DataTypeConversion  OutDataTypeStr=fixdt('ufix32_En0')  LockScale=on
  convert2_1 : DataTypeConversion  OutDataTypeStr=fixdt('ufix32_En0')  ConvertRealWorld=Stored Integer (SI)  LockScale=on
  gain_1 : Gain
  io_delay : xbsIndex_r4/Delay  rst=off  infoeditControl=Selection of Reset will increase slice count due to use of real FFs and instead of SRLs  en=off  latency=0  reg_retiming=on  dbl_ovrd=off  block_type=delay
  reint1 : xbsIndex_r4/Reinterpret  force_arith_type=on  arith_type=Unsigned  force_bin_pt=on  bin_pt=0  block_type=reinterpret
  s_b4a4x1kf_sys3_vacc_tvg0_ins_vect_val_user_data_out : xbsIndex_r4/Gateway In  gui_display_data_type=Fixed-point  arith_type=Unsigned  n_bits=32  bin_pt=0  preci_type=Single  exp_width=8  frac_width=24  rows=1  columns=1  quantization="Round  (unbiased: +/- Inf)"  overflow=Saturate  period=1  UseAsADC=off  ADCChannel='1'  interface=None  automatic_assignment=on  address_offset=hex2dec('00')  intf_name=''  intf_description=''  default_value=0  timing_constraint=None  locs_specified=off  LOCs={}  io_standard={}  inherit_from_input=off  hdl_port=on  dbl_ovrd=off  block_type=gatewayin
  slice_reg : xbsIndex_r4/Slice  nbits=32  boolean_output=off  mode=Lower Bit Location + Width  bit1=0  base1=MSB of Input  bit0=0  base0=LSB of Input  dbl_ovrd=off  block_type=slice
  in_reg : Outport
  wires:
  s_b4a4x1kf_sys3_vacc_tvg0_ins_vect_val_user_data_out/1 -> io_delay/1
  sim_1/1 -> convert1_1/1
  convert1_1/1 -> convert2_1/1
  convert2_1/1 -> gain_1/1
  gain_1/1 -> s_b4a4x1kf_sys3_vacc_tvg0_ins_vect_val_user_data_out/1
  io_delay/1 -> slice_reg/1
  slice_reg/1 -> reint1/1
  reint1/1 -> in_reg/1
